simulink model "Simulateur_palan_version2024"  (R2024b)
settings: Solver=ode4  StartTime=0.0  StopTime=20  RelTol=1e-3
values from neighbouring files (symbols this model uses):
  F = sysd.A    [Script_projet_section2.m]    (also in labo6_simulation.m)
  G = 0.002    [Essai_boucle_ouverte.mat]    (also in PAR_PAL1_IDENT.m; Script_projet_section2.m = sysd.B; labo6_simulation.m = sysd.B; mncarres_incomplet.m)
  Kr = [0.1 0 0 0]    [Essai_boucle_ouverte.mat]    (also in Script_projet_section2.m = [9.0560    4.5832  -13.7344    0.1]; labo6_simulation.m = [9.9952 2.8361 -8.7562 1.2009])
  L = 0.1    [ETAT_PAL_IDENT.m]    (also in Essai_boucle_ouverte.mat; Script_projet_section2.m = 1; labo6_simulation.m; p1_cre_18V_droite_0m.mat = 0)
  xd = [0.5 0 0 0]    [Essai_boucle_ouverte.mat]    (also in Script_projet_section2.m = [0.5 0 0 0]'; labo6_simulation.m = [0.5 0 0 0]')
settings Model: Creator=Ale  LastModifiedBy=justi
settings ConfigComp: CovBoundaryAbsTol=1.0e-5

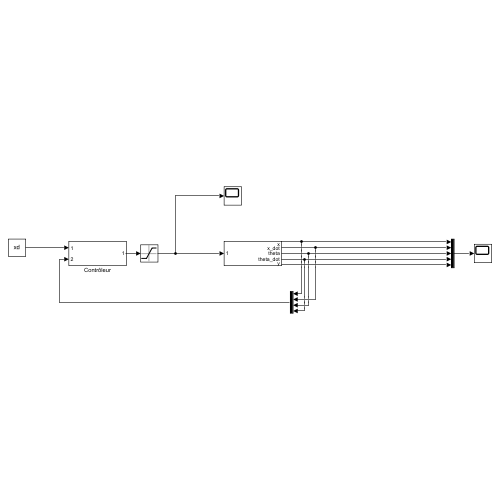
[thumbnail: Simulink's stored preview of the top-level diagram]
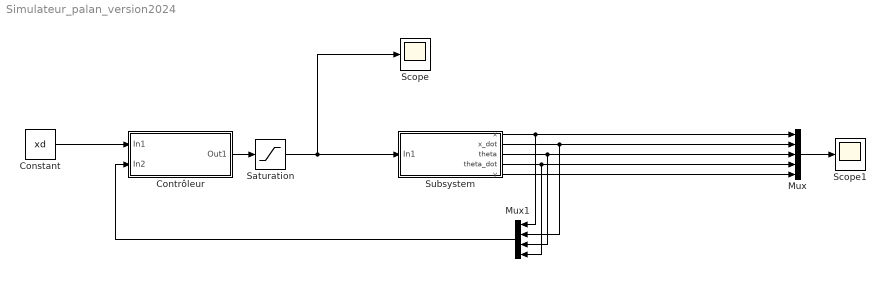
== system Simulateur_palan_version2024 ==
  Constant : Constant  Value=xd
  Contrôleur : Subsystem
  Mux : Mux  Inputs=5
  Mux1 : Mux
  Saturation : Saturate  UpperLimit=24  LowerLimit=-24
  Scope : Scope
  Scope1 : Scope
  Subsystem : Subsystem
  wires:
  Subsystem/1(x) -> Mux1/1, Mux/1
  Subsystem/2(x_dot) -> Mux1/2, Mux/2
  Subsystem/3(theta) -> Mux1/3, Mux/3
  Subsystem/4(theta_dot) -> Mux1/4, Mux/4
  Subsystem/5(y) -> Mux/5
  Mux/1 -> Scope1/1
  Constant/1 -> Contrôleur/1(In1)
  Mux1/1 -> Contrôleur/2(In2)
  Contrôleur/1(Out1) -> Saturation/1
  Saturation/1 -> Scope/1, Subsystem/1(In1)

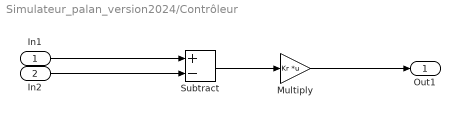
== system Simulateur_palan_version2024/Contrôleur ==
  In1 : Inport
  In2 : Inport  Port=2
  Multiply : Gain  Gain=Kr  Multiplication=Matrix(K*u)
  Subtract : Sum  Inputs=+-
  Out1 : Outport
  wires:
  In1/1 -> Subtract/1
  In2/1 -> Subtract/2
  Subtract/1 -> Multiply/1
  Multiply/1 -> Out1/1

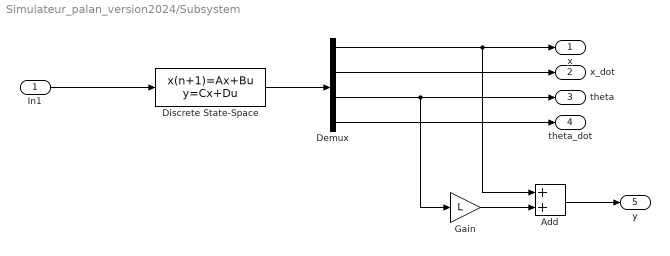
== system Simulateur_palan_version2024/Subsystem ==
  In1 : Inport
  Add : Sum
  Demux : Demux
  Discrete State-Space : DiscreteStateSpace  A=F  B=G  C=[1 0 0 0;0 1 0 0; 0 0 1 0; 0 0 0 1]  D=[0;0;0;0]  SampleTime=-1
  Gain : Gain  Gain=L
  x : Outport
  x_dot : Outport  Port=2
  theta : Outport  Port=3
  theta_dot : Outport  Port=4
  y : Outport  Port=5
  wires:
  Demux/2 -> x_dot/1
  Demux/1 -> x/1, Add/1
  Demux/4 -> theta_dot/1
  Demux/3 -> theta/1, Gain/1
  Gain/1 -> Add/2
  Add/1 -> y/1
  In1/1 -> Discrete State-Space/1
  Discrete State-Space/1 -> Demux/1
